simulink model "C_filter"  (R2024b)
settings: Solver=FixedStepAuto  StartTime=0.0  StopTime=inf  FixedStep=0.01  RelTol=1e-3  EnableMultiTasking=on
libraries: px4Sensorslib x4
settings Model: ExtModeTrigDuration=10  Creator=xippa  LastModifiedBy=xippa
settings SolverCC: PositivePriorityOrder=on
settings OptimizationCC: EnhancedBackFolding=on  PassReuseOutputArgsAs=Individual arguments  ZeroExternalMemoryAtStartup=off  ZeroInternalMemoryAtStartup=off  MaxStackSize=64  OptimizeBlockOrder=speed  DifferentSizesBufferReuse=on  OptimizationCustomize=off  EfficientTunableParamExpr=on
settings DebuggingCC: ParameterTunabilityLossMsg=error
settings HardwareCC: ProdBitPerPointer=32  ProdBitPerSizeT=32  ProdBitPerPtrDiffT=32  ProdLargestAtomicInteger=Long  ProdLargestAtomicFloat=Double  ProdWordSize=32  ProdLongLongMode=on  ProdHWDeviceType=ARM Compatible->ARM Cortex
settings SFSimCC: MATLABDynamicMemAlloc=off  SimTargetLang=C++
settings RTWCC: Description=Embedded Coder  SystemTargetFile=ert.tlc  HardwareBoard=PX4 Cube Orange  TLCOptions="-aInlineSetEventsForThisBaseRateFcn=TLC_FALSE -aSuppressMultiTaskScheduler=TLC_FALSE  -aRateBasedStepFcn=0"  TemplateMakefile=ert_default_tmf  Toolchain=GNU Tools for PX4 Autopilots  TargetLang=C++
settings CodeAppCC: ForceParamTrailComments=on  IgnoreCustomStorageClasses=off  OperatorAnnotations=on  SimulinkDataObjDesc=on  SFDataObjDesc=on  InsertBlockDesc=on
settings ERTTargetCC: ExtModeTransport=3  ExtModeStaticAlloc=on  ExtModeStaticAllocSize=1024  ExtModeMexFile=ext_xcp  ExtModeIntrfLevel=Level2 - Open  InlinedParameterPlacement=Hierarchical

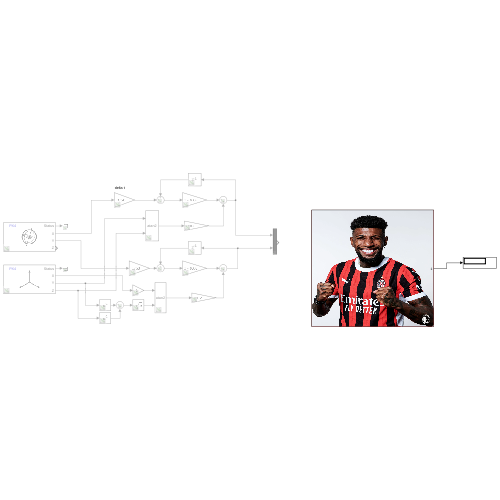
[thumbnail: Simulink's stored preview of the top-level diagram]
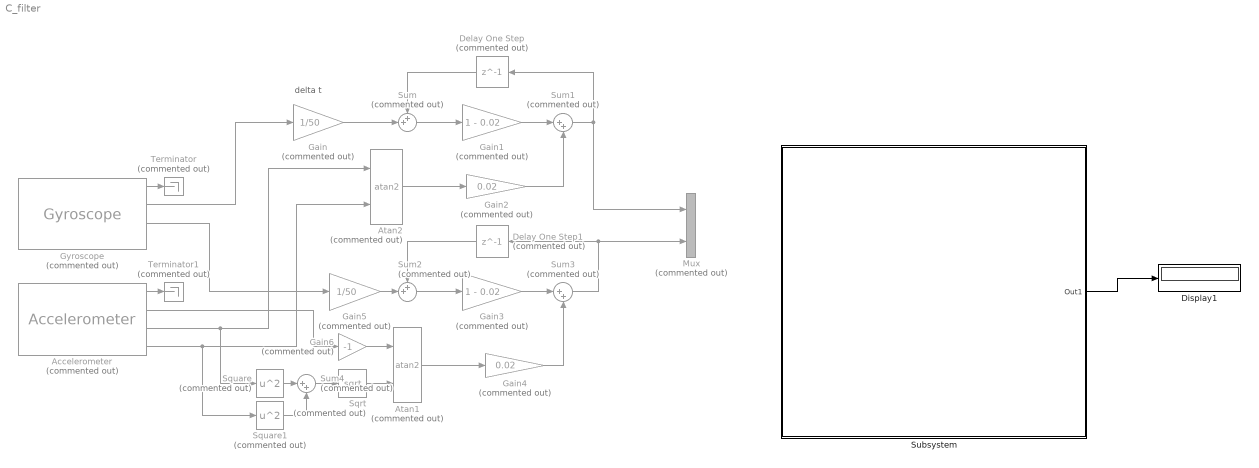
== system C_filter ==
  note: delta t
  Accelerometer : px4Sensorslib/Accelerometer  Commented=on  uorbTimeStamp=off  BlockingMode=off  BlockTimeout=1e-3  sampleTime=1/50
  Atan1 : Trigonometry  Commented=on  Operator=atan2
  Atan2 : Trigonometry  Commented=on  Operator=atan2
  Delay One Step : Delay  Commented=on  DelayLength=1
  Delay One Step1 : Delay  Commented=on  DelayLength=1
  Display1 : Display
  Gain : Gain  Commented=on  Gain=1/50
  Gain1 : Gain  Commented=on  Gain=1 - 0.02
  Gain2 : Gain  Commented=on  Gain=0.02
  Gain3 : Gain  Commented=on  Gain=1 - 0.02
  Gain4 : Gain  Commented=on  Gain=0.02
  Gain5 : Gain  Commented=on  Gain=1/50
  Gain6 : Gain  Commented=on  Gain=-1
  Gyroscope : px4Sensorslib/Gyroscope  Commented=on  uorbTimeStamp=off  BlockingMode=off  BlockTimeout=1e-3  sampleTime=1/50
  Mux : Mux  Commented=on  Inputs=2
  Sqrt : Sqrt  Commented=on
  Square : Math  Commented=on  Operator=square
  Square1 : Math  Commented=on  Operator=square
  Subsystem : Subsystem
      mask Display: image('Screenshot 2024-11-06 175715.png');
  Sum : Sum  Commented=on  Inputs=++|
  Sum1 : Sum  Commented=on  Inputs=|++
  Sum2 : Sum  Commented=on  Inputs=++|
  Sum3 : Sum  Commented=on  Inputs=|++
  Sum4 : Sum  Commented=on  Inputs=|++
  Terminator : Terminator  Commented=on
  Terminator1 : Terminator  Commented=on
  wires:
  Gyroscope/1 -> Terminator/1
  Accelerometer/1 -> Terminator1/1
  Gyroscope/2 -> Gain/1
  Gain/1 -> Sum/2
  Sum/1 -> Gain1/1
  Gain1/1 -> Sum1/1
  Sum1/1 -> Mux/1, Delay One Step/1
  Delay One Step/1 -> Sum/1
  Accelerometer/3 -> Square/1, Atan2/1
  Accelerometer/4 -> Square1/1, Atan2/2
  Atan2/1 -> Gain2/1
  Gain2/1 -> Sum1/2
  Atan1/1 -> Gain4/1
  Gain4/1 -> Sum3/2
  Delay One Step1/1 -> Sum2/1
  Sum3/1 -> Delay One Step1/1, Mux/2
  Sum2/1 -> Gain3/1
  Gain3/1 -> Sum3/1
  Gain5/1 -> Sum2/2
  Gyroscope/3 -> Gain5/1
  Accelerometer/2 -> Gain6/1
  Gain6/1 -> Atan1/1
  Square/1 -> Sum4/1
  Square1/1 -> Sum4/2
  Sum4/1 -> Sqrt/1
  Sqrt/1 -> Atan1/2
  Subsystem/1(Out1) -> Display1/1

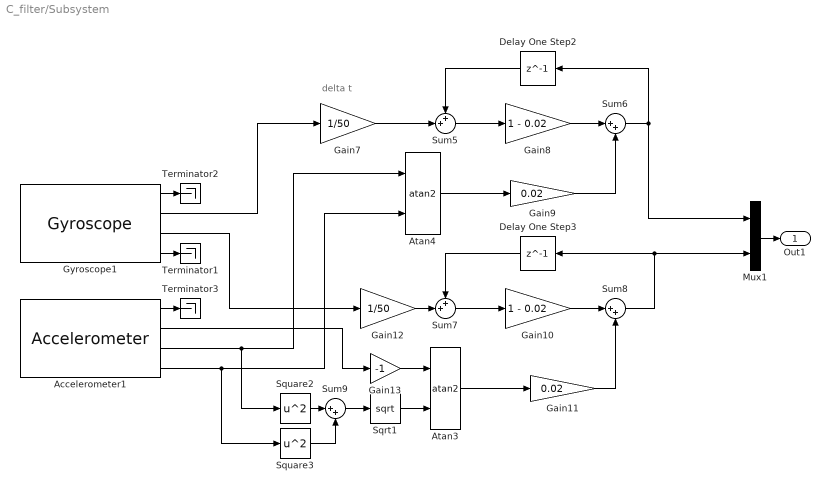
== system C_filter/Subsystem ==
  note: delta t
  Accelerometer1 : px4Sensorslib/Accelerometer  uorbTimeStamp=off  BlockingMode=off  BlockTimeout=1e-3  sampleTime=1/50
  Atan3 : Trigonometry  Operator=atan2
  Atan4 : Trigonometry  Operator=atan2
  Delay One Step2 : Delay  DelayLength=1
  Delay One Step3 : Delay  DelayLength=1
  Gain10 : Gain  Gain=1 - 0.02
  Gain11 : Gain  Gain=0.02
  Gain12 : Gain  Gain=1/50
  Gain13 : Gain  Gain=-1
  Gain7 : Gain  Gain=1/50
  Gain8 : Gain  Gain=1 - 0.02
  Gain9 : Gain  Gain=0.02
  Gyroscope1 : px4Sensorslib/Gyroscope  uorbTimeStamp=off  BlockingMode=off  BlockTimeout=1e-3  sampleTime=1/50
  Mux1 : Mux  Inputs=2
  Sqrt1 : Sqrt
  Square2 : Math  Operator=square
  Square3 : Math  Operator=square
  Sum5 : Sum  Inputs=++|
  Sum6 : Sum  Inputs=|++
  Sum7 : Sum  Inputs=++|
  Sum8 : Sum  Inputs=|++
  Sum9 : Sum  Inputs=|++
  Terminator1 : Terminator
  Terminator2 : Terminator
  Terminator3 : Terminator
  Out1 : Outport
  wires:
  Delay One Step3/1 -> Sum7/1
  Gain10/1 -> Sum8/1
  Sum9/1 -> Sqrt1/1
  Accelerometer1/3 -> Square2/1, Atan4/1
  Sum7/1 -> Gain10/1
  Accelerometer1/4 -> Square3/1, Atan4/2
  Gain9/1 -> Sum6/2
  Sum5/1 -> Gain8/1
  Mux1/1 -> Out1/1
  Atan3/1 -> Gain11/1
  Square3/1 -> Sum9/2
  Atan4/1 -> Gain9/1
  Gyroscope1/3 -> Gain12/1
  Square2/1 -> Sum9/1
  Sum6/1 -> Mux1/1, Delay One Step2/1
  Gain11/1 -> Sum8/2
  Sqrt1/1 -> Atan3/2
  Accelerometer1/2 -> Gain13/1
  Delay One Step2/1 -> Sum5/1
  Gain13/1 -> Atan3/1
  Gain12/1 -> Sum7/2
  Gyroscope1/4 -> Terminator1/1
  Accelerometer1/1 -> Terminator3/1
  Sum8/1 -> Delay One Step3/1, Mux1/2
  Gyroscope1/1 -> Terminator2/1
  Gain8/1 -> Sum6/1
  Gyroscope1/2 -> Gain7/1
  Gain7/1 -> Sum5/2
